simulink model "ex1"  (R2025b)
settings: Solver=VariableStepAuto  StartTime=0.0  StopTime=1.3  FixedStep=1e-4  RelTol=1e-4
values from neighbouring files (symbols this model uses):
  al = ap * 10    [sim3.m]
  kip = ap*ap/psi_nominal    [sim3.m]
  kpp = 2*ap/psi_nominal    [sim3.m]
  Te_nominal = Te_base * k    [sim3.m]
  V_base = sqrt(2) * K * (V_n)    [sim3.m]
  w_base = 2*pi*f_base    (= 314.159265359)    [sim3.m]
settings Model: Creator=Dimitris  LastModifiedBy=Dimitris

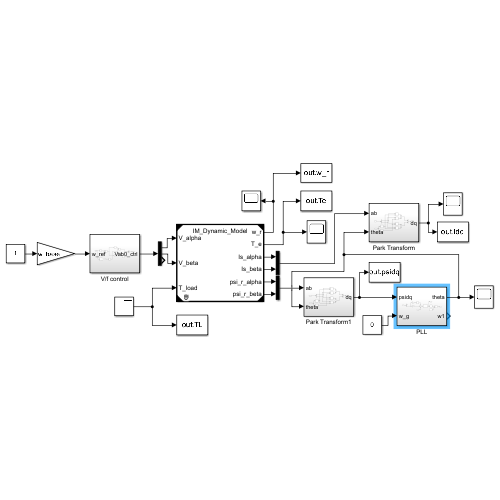
[thumbnail: Simulink's stored preview of the top-level diagram]
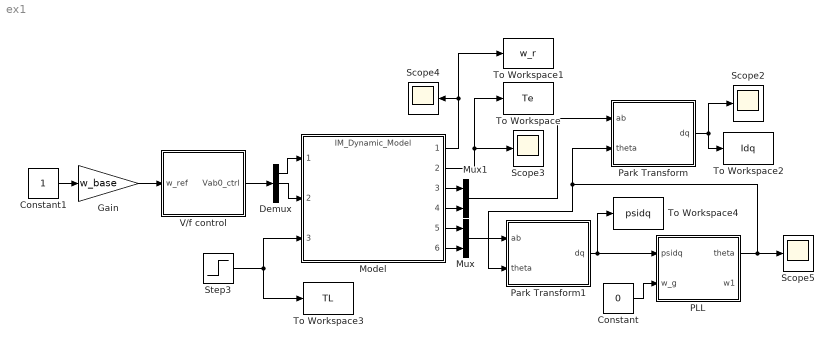
== system ex1 ==
  Constant : Constant  Value=0
  Constant1 : Constant
  Demux : Demux  Outputs=3
  Gain : Gain  Gain=w_base
  Model : ModelReference  ModelNameDialog=IM_Dynamic_Model.slxp  ModelReferenceVersion=1.0  CopyOfModelProtected=on
  Mux : Mux  Inputs=2
  Mux1 : Mux  Inputs=2
  PLL : Subsystem
  Park Transform : Subsystem
  Park Transform1 : Subsystem
  Scope{2..5} (4 alike) : Scope
      Scope2 settings: ActiveDisplayYMinimum=-26.634031862418254  ActiveDisplayYMaximum=26.987549785949923  DataLoggingVariableName=ScopeData2
      Scope3 settings: ActiveDisplayYMinimum=-18.069742755359798  ActiveDisplayYMaximum=33.730348086137596  DataLoggingVariableName=ScopeData3
      Scope4 settings: ActiveDisplayYMinimum=-1  ActiveDisplayYMaximum=1  DataLoggingVariableName=ScopeData4
      Scope5 settings: ActiveDisplayYMinimum=-0.78539816339744806  ActiveDisplayYMaximum=7.0685834705770345  DataLoggingVariableName=ScopeData5
  Step3 : Step  Time=0.7  After=Te_nominal/2  SampleTime=0
  To Workspace : ToWorkspace  VariableName=Te  SaveFormat=Timeseries  SampleTime=-1
  To Workspace1 : ToWorkspace  VariableName=w_r  SaveFormat=Timeseries  SampleTime=-1
  To Workspace2 : ToWorkspace  VariableName=Idq  SaveFormat=Timeseries  SampleTime=-1
  To Workspace3 : ToWorkspace  VariableName=TL  SaveFormat=Timeseries  SampleTime=-1
  To Workspace4 : ToWorkspace  VariableName=psidq  SaveFormat=Timeseries  SampleTime=-1
  V/f control : Subsystem
  wires:
  Model/2 -> To Workspace/1, Scope3/1
  Gain/1 -> V/f control/1(w_ref)
  Step3/1 -> To Workspace3/1, Model/3
  Demux/2 -> Model/2
  Demux/1 -> Model/1
  Model/5 -> Mux/1
  Model/6 -> Mux/2
  PLL/1(theta) -> Scope5/1, Park Transform1/2(theta), Park Transform/2(theta)
  V/f control/1(Vab0_ctrl) -> Demux/1
  Model/3 -> Mux1/1
  Model/4 -> Mux1/2
  Mux1/1 -> Park Transform/1(ab)
  Park Transform/1(dq) -> To Workspace2/1, Scope2/1
  Constant1/1 -> Gain/1
  Model/1 -> To Workspace1/1, Scope4/1
  Park Transform1/1(dq) -> PLL/1(psidq), To Workspace4/1
  Mux/1 -> Park Transform1/1(ab)
  Constant/1 -> PLL/2(w_g)

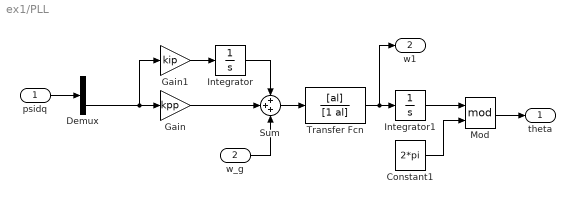
== system ex1/PLL ==
  psidq : Inport
  w_g : Inport  Port=2
  Constant1 : Constant  Value=2*pi
  Demux : Demux  Outputs=2
  Gain : Gain  Gain=kpp
  Gain1 : Gain  Gain=kip
  Integrator : Integrator
  Integrator1 : Integrator
  Mod : Math  Operator=mod
  Sum : Sum  Inputs=+++
  Transfer Fcn : TransferFcn  Numerator=[al]  Denominator=[1 al]
  theta : Outport
  w1 : Outport  Port=2
  wires:
  Gain1/1 -> Integrator/1
  Gain/1 -> Sum/2
  Sum/1 -> Transfer Fcn/1
  Transfer Fcn/1 -> w1/1, Integrator1/1
  Constant1/1 -> Mod/2
  Integrator1/1 -> Mod/1
  Mod/1 -> theta/1
  Demux/2 -> Gain1/1, Gain/1
  psidq/1 -> Demux/1
  Integrator/1 -> Sum/1
  w_g/1 -> Sum/3

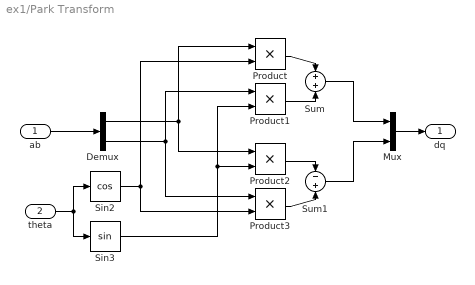
== system ex1/Park Transform ==
  ab : Inport
  theta : Inport  Port=2
  Demux : Demux  Outputs=2
  Mux : Mux  Inputs=2
  Product{,1..3} (4 alike) : Product
  Sin2 : Trigonometry  Operator=cos
  Sin3 : Trigonometry
  Sum : Sum
  Sum1 : Sum  Inputs=-+
  dq : Outport
  wires:
  Sin3/1 -> Product1/2, Product2/2
  Sin2/1 -> Product/2, Product3/2
  theta/1 -> Sin3/1, Sin2/1
  Demux/2 -> Product1/1, Product3/1
  Sum1/1 -> Mux/2
  Sum/1 -> Mux/1
  Demux/1 -> Product2/1, Product/1
  Product2/1 -> Sum1/1
  Product3/1 -> Sum1/2
  Product1/1 -> Sum/2
  Product/1 -> Sum/1
  Mux/1 -> dq/1
  ab/1 -> Demux/1

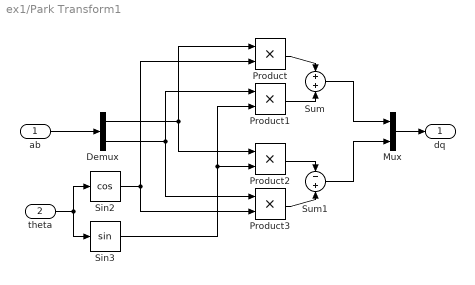
== system ex1/Park Transform1 ==
  ab : Inport
  theta : Inport  Port=2
  Demux : Demux  Outputs=2
  Mux : Mux  Inputs=2
  Product{,1..3} (4 alike) : Product
  Sin2 : Trigonometry  Operator=cos
  Sin3 : Trigonometry
  Sum : Sum
  Sum1 : Sum  Inputs=-+
  dq : Outport
  wires:
  Sin3/1 -> Product1/2, Product2/2
  Sin2/1 -> Product/2, Product3/2
  theta/1 -> Sin3/1, Sin2/1
  Demux/2 -> Product1/1, Product3/1
  Sum1/1 -> Mux/2
  Sum/1 -> Mux/1
  Demux/1 -> Product2/1, Product/1
  Product2/1 -> Sum1/1
  Product3/1 -> Sum1/2
  Product1/1 -> Sum/2
  Product/1 -> Sum/1
  Mux/1 -> dq/1
  ab/1 -> Demux/1

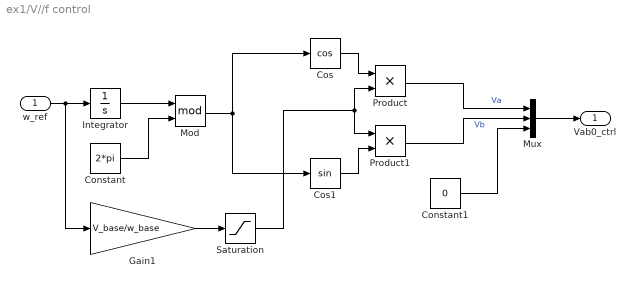
== system ex1/V//f control ==
  w_ref : Inport
  Constant : Constant  Value=2*pi
  Constant1 : Constant  Value=0
  Cos : Trigonometry  Operator=cos
  Cos1 : Trigonometry
  Gain1 : Gain  Gain=V_base/w_base
  Integrator : Integrator
  Mod : Math  Operator=mod
  Mux : Mux  Inputs=3
  Product : Product
  Product1 : Product
  Saturation : Saturate  UpperLimit=V_base  LowerLimit=-V_base
  Vab0_ctrl : Outport
  wires:
  Constant/1 -> Mod/2
  Integrator/1 -> Mod/1
  Cos1/1 -> Product1/2
  Gain1/1 -> Saturation/1
  w_ref/1 -> Gain1/1, Integrator/1
  Mod/1 -> Cos1/1, Cos/1
  Cos/1 -> Product/1
  Saturation/1 -> Product1/1, Product/2
  Product/1 -> Mux/1  "Va"
  Product1/1 -> Mux/2  "Vb"
  Constant1/1 -> Mux/3
  Mux/1 -> Vab0_ctrl/1
